simulink model "mzSimulation"  (R2026b)
settings: Solver=VariableStepAuto
StartFcn:
  | % ---- Settings (edit these per run) ----
  | gen_dataName = 'A2356run4.mat';              % file inside the Inputs folder
  | gen_outName  = 'R20Round4&5';                % folder inside data/Outputs
  | 
  | % Change these based off of inclination angle/tire type (see Teams)
  | gen_idx50   = 5006:6220;
  | gen_idx100  = 7491:8645;
  | gen_idx150  = 3754:4937;
  | gen_idx200  = 2546:3667;
  | gen_idx250a = 1:2484;
  | gen_idx250b = 6255:7418;
  | 
  | % ---- Paths relative to the .slx so the folder can be moved anywhere ----
  | gen_modelDir = fileparts(get_param(bdroot, 'FileName'));
  | gen_dataFile = fullfile(gen_modelDir, 'Inputs', gen_dataName);
  | gen_outDir   = fullfile(gen_modelDir, 'data', 'Outputs', gen_outName);
  | if ~exist(gen_outDir, 'dir'), mkdir(gen_outDir); end
  | 
  | % ---- Load and build the table ----
  | gen_cur = load(gen_dataFile);
  | disp("Loaded " + gen_dataFile);
  | 
  | gen_T = table(gen_cur.AMBTMP, gen_cur.ET, gen_cur.FX, gen_cur.FY, gen_cur.FZ, gen_cur.IA, gen_cur.MX, gen_cur.MZ, ...
  |     gen_cur.N, gen_cur.NFX, gen_cur.NFY, gen_cur.P, gen_cur.RE, gen_cur.RL, gen_cur.RST, ...
  |     gen_cur.SA, gen_cur.SL, gen_cur.SR, gen_cur.TSTC, gen_cur.TSTI, gen_cur.TSTO, gen_cur.V, ...
  |     'VariableNames', {'AmbientRoomTemperature', 'ElapsedTime', 'LongitudinalForce', 'LateralForce', ...
  |     'NormalForce', 'InclinationAngle', 'OverturningMoment', 'AligningTorque', 'WheelRotationalSpeed', ...
  |     'NormalizedLongitudinalForce_FX_FZ', 'NormalizedLateralForce_FY_FZ', 'TirePressure', ...
  |     'EffectiveRadius', 'LoadedRadius', 'RoadSurfaceTemperature', 'SlipAngle', 'SlipRatioTextbook', ...
  |     'SlipRatioBasedOnRL', 'TireSurfaceTemperature_Center', 'TireSurfaceTemperature_Inboard', ...
  |     'TireSurfaceTemperature_Outboard', 'RoadSpeed'});
  | 
  | gen_n = height(gen_T);
  | gen_T.testid = repmat(string(gen_cur.testid), gen_n, 1);
  | gen_T.tireid = repmat(string(gen_cur.tireid), gen_n, 1);
  | gen_T.Index  = (1:gen_n)';
  | 
  | % ---- Slice by FZ and write CSVs ----
  | gen_sub.FZ50  = gen_T(gen_idx50,  :);
  | gen_sub.FZ100 = gen_T(gen_idx100, :);
  | gen_sub.FZ150 = gen_T(gen_idx150, :);
  | gen_sub.FZ200 = gen_T(gen_idx200, :);
  | gen_sub.FZ250 = [gen_T(gen_idx250a, :); gen_T(gen_idx250b, :)];
  | 
  | gen_names = fieldnames(gen_sub);
  | for gen_i = 1:numel(gen_names)
  |     gen_f = fullfile(gen_outDir, sprintf("R20_FZ_%s.csv", gen_names{gen_i}(3:end)));
  |     writetable(gen_sub.(gen_names{gen_i}), gen_f);
  |     disp("Saved: " + gen_f);
  | end
  | disp("All FZ bin CSV files successfully exported.");
  | 
  | % ---- Organize / filter / plot the IA-4 CSVs ----
  | org_files = dir(fullfile(gen_outDir, "R20MZ_FZ_*_IA-4.csv"));
  | if isempty(org_files)
  |     warning("No IA-4 CSV files found in %s", gen_outDir);
  | end
  | 
  | for org_i = 1:numel(org_files)
  |     org_path = fullfile(org_files(org_i).folder, org_files(org_i).name);
  |     org_T = readtable(org_path);
  | 
  |     org_vars = ["RoadSpeed", "TirePressure", "InclinationAngle", "NormalForce", ...
  |         "SlipAngle", "ElapsedTime", "AligningTorque", "LateralForce", "Index"];
  |     org_T = org_T(:, org_vars);
  | 
  |     org_T.RoadSpeed        = round(org_T.RoadSpeed);
  |     org_T.TirePressure     = floor(org_T.TirePressure);
  |     org_T.InclinationAngle = floor(org_T.InclinationAngle * 10) / 10;
  |     org_T = sortrows(org_T, ["RoadSpeed", "TirePressure", "InclinationAngle"]);
  | 
  |     org_F = org_T(org_T.InclinationAngle == 4 & org_T.RoadSpeed == 25 & org_T.TirePressure == 12, :);
  |     org_F = sortrows(org_F, "ElapsedTime");
  | 
  |     [~, org_name, ~] = fileparts(org_files(org_i).name);
  |     org_outName = sprintf('%s_filtered.csv', org_name);
  |     writetable(org_F, fullfile(gen_outDir, org_outName));
  | 
  |     figure('Name', org_outName, 'NumberTitle', 'off');
  |     plot(org_F.ElapsedTime, org_F.NormalForce,    'b-', 'LineWidth', 1.5); hold on;
  |     plot(org_F.ElapsedTime, org_F.SlipAngle,      'r-', 'LineWidth', 1.5);
  |     plot(org_F.ElapsedTime, org_F.LateralForce,   'g-', 'LineWidth', 1.5);
  |     plot(org_F.ElapsedTime, org_F.AligningTorque, 'y-', 'LineWidth', 1.5);
  |     hold off; grid on;
  |     xlabel('Elapsed Time (s)'); ylabel('Value');
  |     title(strrep(org_outName, '_', '\_'));
  |     legend('Normal Force (N)', 'Slip Angle (deg)', 'Lateral Force (N)', 'Aligning Torque', 'Location', 'best');
  |     saveas(gcf, fullfile(gen_outDir, sprintf('%s_diagnostic_plot.png', org_name)));
  |     % close(gcf);
  | end
  | disp("Organize step complete.");
  | 
  | % ---- Combine the filtered IA-4 CSVs into one file ----
  | comb_files = dir(fullfile(gen_outDir, 'R20MZ_FZ_*_IA-4_filtered.csv'));
  | if isempty(comb_files)
  |     warning("No filtered IA-4 CSV files found in %s", gen_outDir);
  | else
  |     comb_T = table();
  |     for comb_i = 1:numel(comb_files)
  |         comb_path = fullfile(comb_files(comb_i).folder, comb_files(comb_i).name);
  |         comb_tmp  = readtable(comb_path);
  |         [~, comb_name, ~] = fileparts(comb_files(comb_i).name);
  |         comb_tmp.SourceFile = repmat({comb_name}, height(comb_tmp), 1);
  |         comb_T = [comb_T; comb_tmp]; %#ok<AGROW>
  |     end
  |     comb_T = sortrows(comb_T, 'NormalForce');
  |     writetable(comb_T, fullfile(gen_outDir, 'R20MZ_combined_IA-4_filtered.csv'));
  |     disp("Combined " + numel(comb_files) + " files into R20MZ_combined_IA-4_filtered.csv");
  | end
  | 
  | % ---- Clean up so nothing is left in the base workspace ----
  | clear gen_* org_* comb_*
settings Model: Creator=ajsau  LastModifiedBy=ajsau

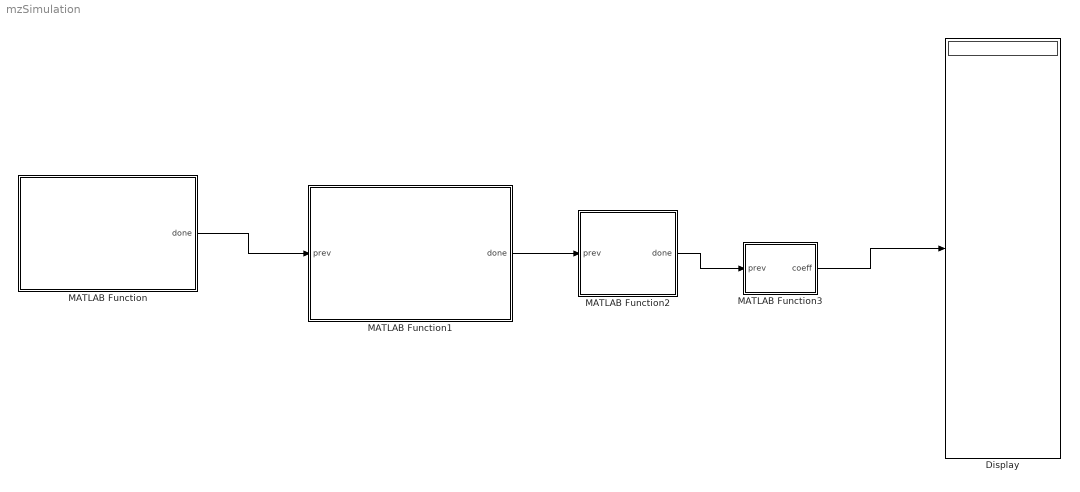
== system mzSimulation ==
  Display : Display
  MATLAB Function : MATLAB Function  TreatAsAtomicUnit=on
  MATLAB Function1 : MATLAB Function  TreatAsAtomicUnit=on
  MATLAB Function2 : MATLAB Function  TreatAsAtomicUnit=on
  MATLAB Function3 : MATLAB Function  TreatAsAtomicUnit=on
  wires:
  MATLAB Function/1(done) -> MATLAB Function1/1(prev)
  MATLAB Function1/1(done) -> MATLAB Function2/1(prev)
  MATLAB Function2/1(done) -> MATLAB Function3/1(prev)
  MATLAB Function3/1(coeff) -> Display/1

== matlab function mzSimulation/MATLAB Function ==
  data: done output
function done = generator()
% BLOCK 1: runs generatorIA0, generatorIA2, generatorIA4. No inputs, one output.
coder.extrinsic('evalin');
done = 0;

persistent hasExecuted
if isempty(hasExecuted)
    hasExecuted = false;
end

if ~hasExecuted
    NL = char(10);
    evalin('base', 'r20_gen_src = '''';');

    % ---------- Entry point: comment out any IA you don't want ----------
    push([ ...
    'function R20Gen()' NL ...
    '    generatorIA0();' NL ...
    '    generatorIA2();' NL ...
    '    generatorIA4();' NL ...
    'end' NL NL ...
    ]);

    % ---------- generatorIA0 ----------
    push([ ...
    'function generatorIA0()' NL ...
    '    dataFile = ''Inputs/A2356run4.mat''; % Change this to round you want' NL ...
    '    outputFolder = ''data/Outputs/R20Round4&5''; % Change this to output you want' NL ...
    '    % Change these based off of inclination angle/tire type (see Teams)' NL ...
    '    idxRange50 = 5006:6220;' NL ...
    '    idxRange100 = 7491:8645;' NL ...
    '    idxRange150 = 3754:4937;' NL ...
    '    idxRange200 = 2546:3667;' NL ...
    '    idxRange250a = 1:2484;' NL ...
    '    idxRange250b = 6255:7418;' NL ...
    '    curFile = load(dataFile);' NL ...
    '    disp("Loaded " + dataFile);' NL ...
    '    runTable = table(curFile.AMBTMP, curFile.ET, curFile.FX, curFile.FY, curFile.FZ, curFile.IA, curFile.MX, curFile.MZ, ...' NL ...
    '        curFile.N, curFile.NFX, curFile.NFY, curFile.P, curFile.RE, curFile.RL, curFile.RST, ...' NL ...
    '        curFile.SA, curFile.SL, curFile.SR, curFile.TSTC, curFile.TSTI, curFile.TSTO, curFile.V, ...' NL ...
    '        ''VariableNames'', {''AmbientRoomTemperature'', ''ElapsedTime'', ''LongitudinalForce'', ''LateralForce'', ...' NL ...
    '        ''NormalForce'', ''InclinationAngle'', ''OverturningMoment'', ''AligningTorque'', ''WheelRotationalSpeed'', ...' NL ...
    '        ''NormalizedLongitudinalForce(FX/FZ)'', ''NormalizedLateralForce(FY/FZ)'', ''TirePressure'', ...' NL ...
    '        ''EffectiveRadius'', ''LoadedRadius'', ''RoadSurfaceTemperature'', ''SlipAngle'', ''SlipRatioTextbook'', ...' NL ...
    '        ''SlipRatioBasedOnRL'', ''TireSurfaceTemperature-Center'', ''TireSurfaceTemperature-Inboard'', ...' NL ...
    '        ''TireSurfaceTemperature-Outboard'', ''RoadSpeed''});' NL ...
    ]);
    push([ ...
    '    runTable.testid = repmat(string(curFile.testid), height(runTable), 1);' NL ...
    '    runTable.tireid = repmat(string(curFile.tireid), height(runTable), 1);' NL ...
    '    runTable.Index = (1:height(runTable))'';' NL ...
    '    disp("Run table created with " + height(runTable) + " rows.");' NL ...
    '    subTables = struct();' NL ...
    '    subTables.FZ50 = runTable(idxRange50, :);' NL ...
    '    subTables.FZ100 = runTable(idxRange100, :);' NL ...
    '    subTables.FZ150 = runTable(idxRange150, :);' NL ...
    '    subTables.FZ200 = runTable(idxRange200, :);' NL ...
    '    subTables.FZ250 = [runTable(idxRange250a, :); runTable(idxRange250b, :)];' NL ...
    '    outNames = fieldnames(subTables);' NL ...
    '    for i = 1:numel(outNames)' NL ...
    '        fname = fullfile(outputFolder, sprintf("R20MZ_FZ_%s_IA-0.csv", outNames{i}(3:end)));' NL ...
    '        writetable(subTables.(outNames{i}), fname);' NL ...
    '        disp("Saved: " + fname);' NL ...
    '    end' NL ...
    '    disp("All FZ bin CSV files successfully exported.");' NL ...
    'end' NL NL ...
    ]);

    % ---------- generatorIA2 ----------
    push([ ...
    'function generatorIA2()' NL ...
    '    dataFile = ''Inputs/A2356run4.mat''; % Change this to round you want' NL ...
    '    outputFolder = ''data/Outputs/R20Round4&5''; % Change this to output you want' NL ...
    '    % Change these based off of inclination angle/tire type (see Teams)' NL ...
    '    idxRange50 = 11224:12388;' NL ...
    '    idxRange100 = 13714:14938;' NL ...
    '    idxRange150 = 9977:11183;' NL ...
    '    idxRange200 = 8733:9910;' NL ...
    '    idxRange250a = 12470:13695;' NL ...
    '    %idxRange250b = 6255:7418;' NL ...
    '    curFile = load(dataFile);' NL ...
    '    disp("Loaded " + dataFile);' NL ...
    '    runTable = table(curFile.AMBTMP, curFile.ET, curFile.FX, curFile.FY, curFile.FZ, curFile.IA, curFile.MX, curFile.MZ, ...' NL ...
    '        curFile.N, curFile.NFX, curFile.NFY, curFile.P, curFile.RE, curFile.RL, curFile.RST, ...' NL ...
    '        curFile.SA, curFile.SL, curFile.SR, curFile.TSTC, curFile.TSTI, curFile.TSTO, curFile.V, ...' NL ...
    '        ''VariableNames'', {''AmbientRoomTemperature'', ''ElapsedTime'', ''LongitudinalForce'', ''LateralForce'', ...' NL ...
    '        ''NormalForce'', ''InclinationAngle'', ''OverturningMoment'', ''AligningTorque'', ''WheelRotationalSpeed'', ...' NL ...
    '        ''NormalizedLongitudinalForce(FX/FZ)'', ''NormalizedLateralForce(FY/FZ)'', ''TirePressure'', ...' NL ...
    '        ''EffectiveRadius'', ''LoadedRadius'', ''RoadSurfaceTemperature'', ''SlipAngle'', ''SlipRatioTextbook'', ...' NL ...
    '        ''SlipRatioBasedOnRL'', ''TireSurfaceTemperature-Center'', ''TireSurfaceTemperature-Inboard'', ...' NL ...
    '        ''TireSurfaceTemperature-Outboard'', ''RoadSpeed''});' NL ...
    ]);
    push([ ...
    '    runTable.testid = repmat(string(curFile.testid), height(runTable), 1);' NL ...
    '    runTable.tireid = repmat(string(curFile.tireid), height(runTable), 1);' NL ...
    '    runTable.Index = (1:height(runTable))'';' NL ...
    '    disp("Run table created with " + height(runTable) + " rows.");' NL ...
    '    subTables = struct();' NL ...
    '    subTables.FZ50 = runTable(idxRange50, :);' NL ...
    '    subTables.FZ100 = runTable(idxRange100, :);' NL ...
    '    subTables.FZ150 = runTable(idxRange150, :);' NL ...
    '    subTables.FZ200 = runTable(idxRange200, :);' NL ...
    '    subTables.FZ250 = runTable(idxRange250a, :);' NL ...
    '    outNames = fieldnames(subTables);' NL ...
    '    for i = 1:numel(outNames)' NL ...
    '        fname = fullfile(outputFolder, sprintf("R20MZ_FZ_%s_IA-2.csv", outNames{i}(3:end)));' NL ...
    '        writetable(subTables.(outNames{i}), fname);' NL ...
    '        disp("Saved: " + fname);' NL ...
    '    end' NL ...
    '    disp("All FZ bin CSV files successfully exported.");' NL ...
    'end' NL NL ...
    ]);

    % ---------- generatorIA4 ----------
    push([ ...
    'function generatorIA4' NL ...
    '    dataFile = ''Inputs/A2356run4.mat''; % Change this to round you want' NL ...
    '    outputFolder = ''data/Outputs/R20Round4&5''; % Change this to output you want' NL ...
    '    % Change these based off of inclination angle/tire type (see Teams)' NL ...
    '    idxRange50 = 17450:18674;' NL ...
    '    idxRange100 = 19942:21169;' NL ...
    '    idxRange150 = 16205:17419;' NL ...
    '    idxRange200 = 14961:16162;' NL ...
    '    idxRange250a = 18696:19922;' NL ...
    '    %idxRange250b = 26177:27399;' NL ...
    '    curFile = load(dataFile);' NL ...
    '    disp("Loaded " + dataFile);' NL ...
    '    runTable = table(curFile.AMBTMP, curFile.ET, curFile.FX, curFile.FY, curFile.FZ, curFile.IA, curFile.MX, curFile.MZ, ...' NL ...
    '        curFile.N, curFile.NFX, curFile.NFY, curFile.P, curFile.RE, curFile.RL, curFile.RST, ...' NL ...
    '        curFile.SA, curFile.SL, curFile.SR, curFile.TSTC, curFile.TSTI, curFile.TSTO, curFile.V, ...' NL ...
    '        ''VariableNames'', {''AmbientRoomTemperature'', ''ElapsedTime'', ''LongitudinalForce'', ''LateralForce'', ...' NL ...
    '        ''NormalForce'', ''InclinationAngle'', ''OverturningMoment'', ''AligningTorque'', ''WheelRotationalSpeed'', ...' NL ...
    '        ''NormalizedLongitudinalForce(FX/FZ)'', ''NormalizedLateralForce(FY/FZ)'', ''TirePressure'', ...' NL ...
    '        ''EffectiveRadius'', ''LoadedRadius'', ''RoadSurfaceTemperature'', ''SlipAngle'', ''SlipRatioTextbook'', ...' NL ...
    '        ''SlipRatioBasedOnRL'', ''TireSurfaceTemperature-Center'', ''TireSurfaceTemperature-Inboard'', ...' NL ...
    '        ''TireSurfaceTemperature-Outboard'', ''RoadSpeed''});' NL ...
    ]);
    push([ ...
    '    runTable.testid = repmat(string(curFile.testid), height(runTable), 1);' NL ...
    '    runTable.tireid = repmat(string(curFile.tireid), height(runTable), 1);' NL ...
    '    runTable.Index = (1:height(runTable))'';' NL ...
    '    disp("Run table created with " + height(runTable) + " rows.");' NL ...
    '    subTables = struct();' NL ...
    '    subTables.FZ50 = runTable(idxRange50, :);' NL ...
    '    subTables.FZ100 = runTable(idxRange100, :);' NL ...
    '    subTables.FZ150 = runTable(idxRange150, :);' NL ...
    '    subTables.FZ200 = runTable(idxRange200, :);' NL ...
    '    subTables.FZ250 = runTable(idxRange250a, :);' NL ...
    '    outNames = fieldnames(subTables);' NL ...
    '    for i = 1:numel(outNames)' NL ...
    '        fname = fullfile(outputFolder, sprintf("R20MZ_FZ_%s_IA-4.csv", outNames{i}(3:end)));' NL ...
    '        writetable(subTables.(outNames{i}), fname);' NL ...
    '        disp("Saved: " + fname);' NL ...
    '    end' NL ...
    '    disp("All FZ bin CSV files successfully exported.");' NL ...
    'end' NL ...
    ]);

    % ---------- Write the temp file and run it ----------
    evalin('base', [ ...
        'r20_dir = fullfile(tempdir, ''R20Pipeline_gen''); ' ...
        'if ~exist(r20_dir, ''dir''), mkdir(r20_dir); end; ' ...
        'r20_fid = fopen(fullfile(r20_dir, ''R20Gen.m''), ''w''); ' ...
        'fwrite(r20_fid, r20_gen_src); fclose(r20_fid); ' ...
        'addpath(r20_dir); rehash; clear R20Gen; ' ...
        'R20Gen(); ' ...
        'clear r20_gen_src r20_gen_chunk r20_dir r20_fid;' ...
    ]);

    hasExecuted = true;
end

done = 1;
end

function push(chunk)
coder.extrinsic('assignin', 'evalin');
assignin('base', 'r20_gen_chunk', chunk);
evalin('base', 'r20_gen_src = [r20_gen_src r20_gen_chunk];');
end

== matlab function mzSimulation/MATLAB Function2 ==
  data: prev input; done output
function done = combine(prev)
% BLOCK 3: combines the filtered IA-4 CSVs. Input 'prev' is the done output of the organize block.
coder.extrinsic('evalin');
done = 0;

persistent hasExecuted
if isempty(hasExecuted)
    hasExecuted = false;
end

if prev > 0 && ~hasExecuted
    NL = char(10);
    evalin('base', 'r20_comb_src = '''';');

    push([ ...
        'function R20Comb()' NL ...
        '    combiner();' NL ...
        'end' NL NL ...
        ]);

    % ---------- combiner ----------
    push([ ...
        'function combiner()' NL ...
        '    dataFolder = ''data/Outputs/R20Round4&5'';' NL ...
        '    filteredFiles = dir(fullfile(dataFolder, ''R20MZ_FZ_*_IA-4_filtered.csv''));' NL ...
        '    combinedTable = table();' NL ...
        '    for i = 1:numel(filteredFiles)' NL ...
        '        curFile = fullfile(filteredFiles(i).folder, filteredFiles(i).name);' NL ...
        '        disp("Adding " + filteredFiles(i).name);' NL ...
        '        tempTable = readtable(curFile);' NL ...
        '        [~, name, ~] = fileparts(filteredFiles(i).name);' NL ...
        '        tempTable.SourceFile = repmat({name}, height(tempTable), 1);' NL ...
        '        combinedTable = [combinedTable; tempTable];' NL ...
        '    end' NL ...
        '    combinedTable = sortrows(combinedTable, ''NormalForce'');' NL ...
        '    outPath = fullfile(dataFolder, ''R20MZ_combined_IA-4_filtered.csv'');' NL ...
        '    writetable(combinedTable, outPath);' NL ...
        '    disp("Combined filtered data saved as: " + outPath);' NL ...
        'end' NL ...
        ]);

    evalin('base', [ ...
        'r20_dir = fullfile(tempdir, ''R20Pipeline_gen''); ' ...
        'if ~exist(r20_dir, ''dir''), mkdir(r20_dir); end; ' ...
        'r20_fid = fopen(fullfile(r20_dir, ''R20Comb.m''), ''w''); ' ...
        'fwrite(r20_fid, r20_comb_src); fclose(r20_fid); ' ...
        'addpath(r20_dir); rehash; clear R20Comb; ' ...
        'R20Comb(); ' ...
        'clear r20_comb_src r20_comb_chunk r20_dir r20_fid;' ...
        ]);

    hasExecuted = true;
end

if hasExecuted
    done = 1;
end
end

function push(chunk)
coder.extrinsic('assignin', 'evalin');
assignin('base', 'r20_comb_chunk', chunk);
evalin('base', 'r20_comb_src = [r20_comb_src r20_comb_chunk];');
end

== matlab function mzSimulation/MATLAB Function3 ==
  data: prev input; coeff output
function coeff = optimize(prev)
% BLOCK 4: runs the Pacejka Mz optimizer. Input 'prev' is the done output of the combine block.
% Outputs: done (scalar), Q (1x24 optimized coefficients) -> wire Q to a Display block.
coder.extrinsic('evalin');

persistent hasExecuted Qsaved
if isempty(hasExecuted)
    hasExecuted = false;
    Qsaved = zeros(1,24);
end

if prev > 0 && ~hasExecuted
    NL = char(10);
    evalin('base', 'r20_opt_src = '''';');

    push([ ...
    'function Q = R20Opt()' NL ...
    '    Q = R20_optimizer();' NL ...
    'end' NL NL ...
    ]);

    % ---------- R20_optimizer (nested function kept intact) ----------
    push([ ...
    'function POptimization = R20_optimizer()' NL ...
    '    data0 = readtable(''data/Outputs/R20Round4&5/R20MZ_combined_IA-0_filtered.csv'');' NL ...
    '    data2 = readtable(''data/Outputs/R20Round4&5/R20MZ_combined_IA-2_filtered.csv'');' NL ...
    '    data4 = readtable(''data/Outputs/R20Round4&5/R20MZ_combined_IA-4_filtered.csv'');' NL ...
    '    data  = [data0; data2; data4];' NL ...
    '    %data = data2;' NL ...
    '' NL ...
    '    %These are different than the FY optimizer so pay attention' NL ...
    '    IA = data{:,3};' NL ...
    '    FZRaw = data{:,4};' NL ...
    '    alpha = data{:,5};' NL ...
    '    MzExperimental = data{:,7};' NL ...
    '    FYExperimental = data{:,8};' NL ...
    '    source = data{:,10};' NL ...
    '' NL ...
    '    FZBins = [50, 100, 150, 200, 250];' NL ...
    '' NL ...
    '    MzAll = [];' NL ...
    '    FYAll = [];' NL ...
    '    FZAll = [];' NL ...
    '    alphaAll = [];' NL ...
    '    IAAll = [];' NL ...
    '' NL ...
    '    for i = 1:numel(FZBins)' NL ...
    '        baseTag = sprintf(''R20MZ_FZ_%d'', FZBins(i));' NL ...
    '        idx = contains(source, [baseTag ''_IA-0_filtered'']) | contains(source, [baseTag ''_IA-2_filtered'']) | contains(source, [baseTag ''_IA-4_filtered'']);' NL ...
    '        MzAll = [MzAll; MzExperimental(idx)];' NL ...
    '        FYAll = [FYAll; FYExperimental(idx)];' NL ...
    '        FZAll = [FZAll; FZBins(i) * ones(sum(idx),1)];' NL ...
    '        alphaAll = [alphaAll; alpha(idx)];' NL ...
    '        IAAll = [IAAll; IA(idx)];' NL ...
    '    end' NL ...
    ]);
    push([ ...
    '    alphaAll = deg2rad(alphaAll);' NL ...
    '    IAAll = deg2rad(IAAll);' NL ...
    '' NL ...
    '    P_fixed = [250, 1.4, 2.4, -0.25, 3, -0.1, -1.5, 0, 0, -30.5, 1.15, 1, 0, 0, -0.128, 0, 0, 0, 1.43];' NL ...
    '    L = ones(1,8);' NL ...
    '' NL ...
    '    % Initial Q guess from Appendix 3' NL ...
    '    Q0 = [0.00276055, 0.00667048, 0.339315, -1.15563, 9.07658, -8.19445, -11.5486, -20.4342, 21.4985, 1.44589, 0.0184206, 0.0141927, 2.24868, -20.2342, 0.337115, -0.984545, -1.95786, 0.122852, -19.6941, -3.55172e-05, -0.000452427, 0.00165919, 0.295113, -0.375074];' NL ...
    '' NL ...
    '    objFun = @(Q) MzExperimental_all(P_fixed, Q, L, FZAll, IAAll, alphaAll, FYAll, MzAll);' NL ...
    '' NL ...
    '    options = optimoptions(''lsqnonlin'', ''Display'', ''iter'', ''MaxFunctionEvaluations'', 30000, ''TolFun'', 1e-8, ''TolX'', 1e-8);' NL ...
    '' NL ...
    '    lb = -Inf(size(Q0));' NL ...
    '    ub = Inf(size(Q0));' NL ...
    '' NL ...
    '    QOptimization = lsqnonlin(objFun, Q0, lb, ub, options);' NL ...
    '' NL ...
    '    disp(''Optimized Q (Mz) Parameters:'');' NL ...
    '    disp(QOptimization);' NL ...
    '' NL ...
    '    MzPredicted = pacejkaMZ(P_fixed, QOptimization, L, FZAll, IAAll, alphaAll, FYAll);' NL ...
    '' NL ...
    '    rmse = sqrt(mean((MzAll - MzPredicted).^2));' NL ...
    '    fprintf(''Overall RMSE (Mz): %.4f Nm\n'', rmse);' NL ...
    '' NL ...
    '    IAValues = [0, 2, 4];' NL ...
    '    colors = lines(numel(FZBins));' NL ...
    ]);
    push([ ...
    '    for k = 1:numel(IAValues)' NL ...
    '        figure;' NL ...
    '        hold on;' NL ...
    '        grid on;' NL ...
    '' NL ...
    '        thisIA = deg2rad(IAValues(k));' NL ...
    '        idxIA = abs(IAAll - thisIA) < 1e-6;' NL ...
    '' NL ...
    '        for i = 1:numel(FZBins)' NL ...
    '            idx = idxIA & (FZAll == FZBins(i));' NL ...
    '' NL ...
    '            scatter(rad2deg(alphaAll(idx)), MzAll(idx), 6, colors(i,:), ''filled'', ''DisplayName'', sprintf(''Exp FZ=%d'', FZBins(i)));' NL ...
    '' NL ...
    '            [alphaSort, ord] = sort(alphaAll(idx));' NL ...
    '            MzFit = pacejkaMZ(P_fixed, QOptimization, L, FZAll(idx), IAAll(idx), alphaSort, FYAll(idx));' NL ...
    '' NL ...
    '            plot(rad2deg(alphaSort), MzFit, ''Color'', colors(i,:), ''LineWidth'', 1.5, ''DisplayName'', sprintf(''Fit FZ=%d'', FZBins(i)));' NL ...
    '        end' NL ...
    '' NL ...
    '        title(sprintf(''Pacejka Mz Fit - IA = %d (RMSE = %.3f)'', IAValues(k), rmse));' NL ...
    '        xlabel(''Slip Angle [deg]'');' NL ...
    '        ylabel(''Aligning Torque Mz'');' NL ...
    '        legend(''Location'', ''best'');' NL ...
    '    end' NL ...
    ]);
    push([ ...
    '    %Brennan''s Graph' NL ...
    '    FZTarget = 200;' NL ...
    '    figure;' NL ...
    '    hold on;' NL ...
    '    grid on;' NL ...
    '    title(sprintf(''Pacejka Mz Fit - FZ = %d flb (All IA)'', FZTarget));' NL ...
    '    xlabel(''Slip Angle [deg]'');' NL ...
    '    ylabel(''Aligning Torque Mz'');' NL ...
    '' NL ...
    '    IAValues = [0, 2, 4];' NL ...
    '    colors = lines(numel(IAValues));' NL ...
    '' NL ...
    '    for k = 1:numel(IAValues)' NL ...
    '        thisIA = deg2rad(IAValues(k));' NL ...
    '        idx = (abs(IAAll - thisIA) < 1e-6) & (FZAll == FZTarget);' NL ...
    '' NL ...
    '        if any(idx)' NL ...
    '' NL ...
    '            scatter(rad2deg(alphaAll(idx)), MzAll(idx), 8, colors(k,:), ''filled'', ''DisplayName'', sprintf(''Exp IA=%d'', IAValues(k)));' NL ...
    '' NL ...
    '            [alphaSort, ord] = sort(alphaAll(idx));' NL ...
    '            MzFit = pacejkaMZ(P_fixed, QOptimization, L, FZAll(idx), IAAll(idx), alphaSort, FYAll(idx));' NL ...
    '            plot(rad2deg(alphaSort), MzFit, ''Color'', colors(k,:), ''LineWidth'', 1.5, ''DisplayName'', sprintf(''Fit IA=%d'', IAValues(k)));' NL ...
    '        end' NL ...
    '    end' NL ...
    ]);
    push([ ...
    '    legend(''Location'', ''best'');' NL ...
    '' NL ...
    '    fprintf(''['');' NL ...
    '    fprintf(''%g, '', QOptimization(1:end-1));' NL ...
    '    fprintf(''%g]\n'', QOptimization(end));' NL ...
    '    POptimization = QOptimization;' NL ...
    '' NL ...
    '    function err = MzExperimental_all(P, Q, L, FZ, IA, alpha, FYexp, MzExp)' NL ...
    '        MzModel = pacejkaMZ(P, Q, L, FZ, IA, alpha, FYexp);' NL ...
    '        err = MzModel - MzExp;' NL ...
    '    end' NL ...
    'end' NL NL ...
    ]);

    % ---------- pacejkaMZ ----------
    push([ ...
    'function MZ0 = pacejkaMZ(P, Q, L, FZ, IA, alpha, FY);' NL ...
    '    %P: The coefficients derived from the FY optimization.' NL ...
    '    %Q: Coefficients being optimized from the textbook' NL ...
    '    %L: Lambdas in the textbook' NL ...
    '    %IA: Inclination Angle' NL ...
    '    %alpha: Slip angle' NL ...
    '    %FY: Cornering Force input (currently not used in this build)' NL ...
    '    Vcx  = 1;' NL ...
    '    Vc   = 1;' NL ...
    '    %Vcy  = 0;' NL ...
    '    Kya  = 1;' NL ...
    '    Kyao = 1;' NL ...
    '    Kyy0 = 1;' NL ...
    '    dfz = (FZ - P(1)) / P(1);' NL ...
    '    Svy = FZ .* (P(16) + P(17) * dfz + (P(18) + P(19) * dfz) .* IA) * L(8) * L(5);' NL ...
    '    Ey = (P(6) + P(7) * dfz) .* (1 - (P(8) + P(9) * IA) .* sign(alpha)) * L(7);' NL ...
    '    Shy = (P(13) + P(14) * dfz + P(15) * IA) * L(6);' NL ...
    '    alphaY = alpha + Shy;' NL ...
    '    Cy = P(2) * L(2);' NL ...
    '    Dy = FZ .* (P(3) + P(4) * dfz) .* (1-P(5) * IA.^2) * L(1);' NL ...
    '    x1 = 2 * atan(FZ / (P(11) * P(1) * L(3)));' NL ...
    '    x2 = P(10) * P(1) * sin(x1) .* (1-P(12) * abs(IA)) * L(4) * L(5);' NL ...
    '    By = x2 ./ (Cy*Dy);' NL ...
    '    x3 = By .* alphaY;' NL ...
    '    FY = Dy .* sin(Cy * atan(x3-Ey .* (x3-atan(x3)))) + Svy;' NL ...
    '    alpha_star = tan(alpha) .* sign(Vcx); %4.E3' NL ...
    '    SHt = Q(1) + (Q(2) .* dfz) + (Q(3) + (Q(4) .* dfz)) .* sin(IA); % 4.E35' NL ...
    '    SHf = Shy + (Svy ./ (Kya + 0.1)); % 4.E38-39' NL ...
    '    alpha_r = alpha_star .* SHf; % 4.E37' NL ...
    '    Br = Q(20) .* By .* Cy; % 4.E45' NL ...
    '    Cr = 1; % 4.E46' NL ...
    ]);
    push([ ...
    '    Dr = FZ .* 8 .* ((Q(21) + (Q(22) .* dfz)) + (Q(23) + (Q(24) .* dfz)) .* sin(IA)) .* (Vcx ./ (Vc + 0.1)); % 4.E47' NL ...
    '    MZr0 = Dr .* cos(Cr .* atan(Br .* alpha_r)); % 4.E36' NL ...
    '    alpha_t = alpha_star + SHt; % 4.E34' NL ...
    '    Bt = (Q(5) + (Q(6) .* dfz) + (Q(7) .* dfz.^2)) .* (1 + (Q(8) .* sin(IA)) + (Q(9) .* abs(sin(IA)))); % 4.E40' NL ...
    '    Ct = Q(10); % 4.E41' NL ...
    '    Dt0 = FZ .* (8 ./ FZ) .* (Q(11) + (Q(12) .* dfz)) .* sign(Vcx); % 4.E42' NL ...
    '    Dt = Dt0 .* (1 + (Q(13) .* sin(IA)) + (Q(14) .* (sin(IA).^2))); % 4.E43' NL ...
    '    Et = (Q(15) + (Q(16) .* dfz) + (Q(17) .* dfz.^2)) .* (1 + (Q(18) + (Q(19) .* sin(IA))) .* (2/pi) .* atan(Bt .* Ct .* alpha_t)); % 4.E44' NL ...
    '    t0 = Dt .* cos(Ct .* atan((Bt .* alpha_t) - Et .* ((Bt .* alpha_t) - atan(Bt .* alpha_t)))) .* (Vcx ./ (Vc + 0.1)); % 4.E33' NL ...
    '    Kzao = Dt0 .* Kyao; % 4.E48' NL ...
    '    Kzyo = FZ .* 8 .* (Q(23) + (Q(24) .* dfz)) - Dt0 .* Kyy0; %4.E49' NL ...
    '    MZ0_prime = -t0 .* FY; % 4.E32' NL ...
    '    MZ0 = MZ0_prime + MZr0; % 4.E31' NL ...
    'end' NL ...
    ]);

    % ---------- Write the temp file, run it, pull Q back ----------
    evalin('base', [ ...
        'r20_dir = fullfile(tempdir, ''R20Pipeline_gen''); ' ...
        'if ~exist(r20_dir, ''dir''), mkdir(r20_dir); end; ' ...
        'r20_fid = fopen(fullfile(r20_dir, ''R20Opt.m''), ''w''); ' ...
        'fwrite(r20_fid, r20_opt_src); fclose(r20_fid); ' ...
        'addpath(r20_dir); rehash; clear R20Opt; ' ...
        'r20_Q = R20Opt();' ...
    ]);

    Qsaved = zeros(1,24);              % must be typed before the extrinsic assignment
    Qsaved = evalin('base', 'r20_Q');  % pull the result back into the block
    evalin('base', 'clear r20_opt_src r20_opt_chunk r20_dir r20_fid r20_Q;');

    hasExecuted = true;
end

coeff = Qsaved;
end

function push(chunk)
coder.extrinsic('assignin', 'evalin');
assignin('base', 'r20_opt_chunk', chunk);
evalin('base', 'r20_opt_src = [r20_opt_src r20_opt_chunk];');
end

== matlab function mzSimulation/MATLAB Function1 ==
  data: prev input; done output
function done = organize(prev)
% BLOCK 2: filters/plots the IA-4 CSVs. Input 'prev' is the done output of the generator block.
coder.extrinsic('evalin');
done = 0;

persistent hasExecuted
if isempty(hasExecuted)
    hasExecuted = false;
end

if prev > 0 && ~hasExecuted
    NL = char(10);
    evalin('base', 'r20_org_src = '''';');

    push([ ...
        'function R20Org()' NL ...
        '    organize();' NL ...
        'end' NL NL ...
        ]);

    % ---------- organize ----------
    push([ ...
        'function organize()' NL ...
        '    dataFolder = ''data/Outputs/R20Round4&5'';' NL ...
        '    csvFiles = dir(fullfile(dataFolder, "R20MZ_FZ_*_IA-4.csv"));' NL ...
        '    for i = 1:numel(csvFiles)' NL ...
        '        curFile = fullfile(csvFiles(i).folder, csvFiles(i).name);' NL ...
        '        disp("Processing " + csvFiles(i).name);' NL ...
        '        table = readtable(curFile);' NL ...
        '        varNames = ["RoadSpeed", "TirePressure", "InclinationAngle", "NormalForce", "SlipAngle", "ElapsedTime", "AligningTorque", "LateralForce", "Index"];' NL ...
        '        table = table(:, varNames);' NL ...
        '        table.RoadSpeed = round(table.RoadSpeed);' NL ...
        '        table.TirePressure = floor(table.TirePressure);' NL ...
        '        table.InclinationAngle = floor(table.InclinationAngle * 10) / 10;' NL ...
        '        table = sortrows(table, ["RoadSpeed", "TirePressure", "InclinationAngle"]);' NL ...
        '        filteredTable = table(table.InclinationAngle == 4 & table.RoadSpeed == 25 & table.TirePressure == 12, :);' NL ...
        '        filteredTable = sortrows(filteredTable, "ElapsedTime");' NL ...
        '        [~, name, ~] = fileparts(csvFiles(i).name);' NL ...
        '        outName = sprintf(''%s_filtered.csv'', name);' NL ...
        '        outPath = fullfile(dataFolder, outName);' NL ...
        '        writetable(filteredTable, outPath);' NL ...
        '        disp("Saved filtered version: " + outName);' NL ...
        '        figure(''Name'', outName, ''NumberTitle'', ''off'');' NL ...
        '        t = filteredTable.ElapsedTime;' NL ...
        '        NF = filteredTable.NormalForce;' NL ...
        '        SA = filteredTable.SlipAngle;' NL ...
        '        CF = filteredTable.LateralForce;' NL ...
        '        MZ = filteredTable.AligningTorque;' NL ...
        ]);
    push([ ...
        '        plot(t, NF, ''b-'', ''LineWidth'', 1.5); hold on;' NL ...
        '        plot(t, SA, ''r-'', ''LineWidth'', 1.5);' NL ...
        '        plot(t, CF, ''g-'', ''LineWidth'', 1.5);' NL ...
        '        plot(t, MZ, ''y-'', ''LineWidth'', 1.5);' NL ...
        '        hold off;' NL ...
        '        grid on;' NL ...
        '        xlabel(''Elapsed Time (s)'');' NL ...
        '        ylabel(''Value'');' NL ...
        '        title(strrep(outName, ''_'', ''\_''));' NL ...
        '        legend(''Normal Force (N)'', ''Slip Angle (deg)'', ''Lateral Force (N)'', ''Aligning Torque'', ''Location'', ''best'');' NL ...
        '        saveas(gcf, fullfile(dataFolder, sprintf(''%s_diagnostic_plot.png'', name)));' NL ...
        '        %close(gcf);' NL ...
        '        disp("Plot saved: " + name + "_diagnostic_plot.png");' NL ...
        '    end' NL ...
        '    disp("All FZ bins processed, filtered, and plotted successfully.");' NL ...
        'end' NL ...
        ]);

    evalin('base', [ ...
        'r20_dir = fullfile(tempdir, ''R20Pipeline_gen''); ' ...
        'if ~exist(r20_dir, ''dir''), mkdir(r20_dir); end; ' ...
        'r20_fid = fopen(fullfile(r20_dir, ''R20Org.m''), ''w''); ' ...
        'fwrite(r20_fid, r20_org_src); fclose(r20_fid); ' ...
        'addpath(r20_dir); rehash; clear R20Org; ' ...
        'R20Org(); ' ...
        'clear r20_org_src r20_org_chunk r20_dir r20_fid;' ...
        ]);

    hasExecuted = true;
end

if hasExecuted
    done = 1;
end
end

function push(chunk)
coder.extrinsic('assignin', 'evalin');
assignin('base', 'r20_org_chunk', chunk);
evalin('base', 'r20_org_src = [r20_org_src r20_org_chunk];');
end
